simulink model "OFDM_Simulink"  (R2024b)
settings: Solver=VariableStepAuto  StartTime=0.0  StopTime=10.0  RelTol=1e-3
settings Model: Creator=Devansh  LastModifiedBy=Devansh

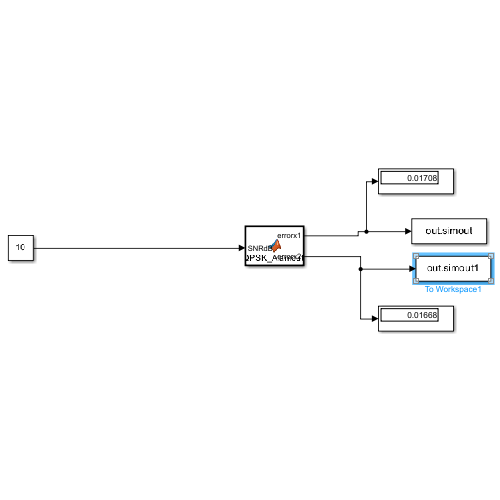
[thumbnail: Simulink's stored preview of the top-level diagram]
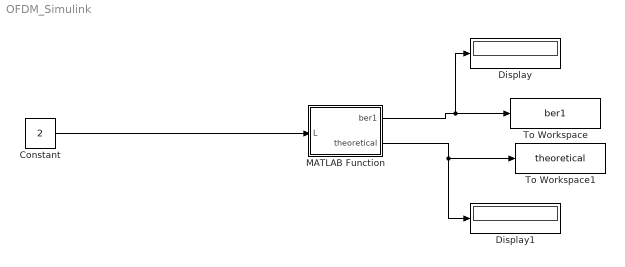
== system OFDM_Simulink ==
  Constant : Constant  Value=2
  Display : Display
  Display1 : Display
  MATLAB Function : MATLAB Function  TreatAsAtomicUnit=on
  To Workspace : ToWorkspace  VariableName=ber1  SampleTime=-1
  To Workspace1 : ToWorkspace  VariableName=theoretical  SampleTime=-1
  wires:
  Constant/1 -> MATLAB Function/1(L)
  MATLAB Function/1(ber1) -> Display/1, To Workspace/1
  MATLAB Function/2(theoretical) -> Display1/1, To Workspace1/1

== matlab function OFDM_Simulink/MATLAB Function ==
  data: L input; ber1 output; theoretical output
function [ber1, theoretical] = OFDM_BPSK(L)

N = 16;
Niter = 1e3;

cp = L-1;

snrdb = 0:3:39;
snrlin = 10.^(snrdb/10);
n_var = 1./snrlin;
nstd = 1./sqrt(2*N*snrlin);

ber = zeros(Niter,length(snrdb));

for iter = 1:Niter

    x1 = randi([0,1],1,N);
    x = 2*x1-1;

    xif = ifft(x,N);
    xcp = [xif(N-cp+1:N),xif];

    for i = 1:length(snrdb)

        h = complex(randn(1,L),randn(1,L))/sqrt(2*L);
        hf = fft(h,N);

        noise = complex(randn(1,N+cp),randn(1,N+cp));

        y = filter(h,1,xcp) + noise*nstd(i);

        yrcp = y(cp+1:N+cp);
        yfrcp = fft(yrcp,N);

        yeq = yfrcp./hf;
        xdet = real(yeq)>0;

        ber(iter,i) = sum(xdet~=x1)/N;

    end
end

ber1 = mean(ber,1);

theoretical = 0.5*(1-sqrt(snrlin./(1+snrlin)));

end
